simulink model "commhdlQPSKTxRxLoopback"  (R2025b)
settings: Solver=FixedStepDiscrete  StartTime=0.0  StopTime=0.03  RelTol=1e-3
PostLoadFcn:
  | hScopeConfig = get_param([gcs '/Receiver/QPSK Rx/Frequency and Time Synchronizer/Symbol Synchronizer/No HDL/QPSK Receiver Eye Diagram'],'ScopeConfiguration');
  | 
  | hScopeConfig.OpenAtSimulationStart = false;
  | hScopeConfig.Visible = false;
  | SamplesPerSymbol = 4;
  | %UpsamplesRx = 1;
  | clear hScopeConfig
InitFcn:
  | % RxAlign decoder latency (flat_simfix): 41 = netlist value used for HDL; set
  | % rxAlignLat = 25 in the base workspace before a model-level simulation.
  | if ~exist('rxAlignLat','var'), rxAlignLat = uint16(41); end
  | commhdlQPSKTxRxModelInit;
  | % Rate bridge: ADRV9002/Jupiter radio runs at 15.36 MHz = 2x the 7.68 MHz
  | % (4 samples/symbol @ Rsym=1.92 MHz) the QPSK Rx requires. The deployed
  | % Receiver must downsample the ADC stream by 2. UpsamplesRx=1 fed the QPSK
  | % Rx 8 sps (2x-upsampled) and broke symbol sync / the loopback bit check.
  | UpsamplesRx = 1;   %% T8 RATE FIX: rail 15.36e6 == ADC bus rate,
  | %% no ingress decimation (was 2 when the rail sat on the 7.68e6 rung)
  | UpsamplesTx = 1;
  | clear simTimingOffset;
StopFcn:
  | if exist('simTimingOffset','var')
  |   disp('Simulation completed');
  |   %QPSKTxRxVerification;
  | end
undefined symbols (not defined in the file or in its folder): Add, Config, fsym, randsrc, RandStream, Rsym, rxAlignLat, Shift
libraries: hdlsllib x141, simulink x45, dspsigops x30, dsphdlfiltering2 x6, dsphdlsigops2 x4, dsphdlmathfun2 x4, commdigbbndpm3 x4, dspmlti4 x2, commchan3 x1, commrflib2 x1, commcnvcod2 x1
(part 9 of 9)

== matlab function commhdlQPSKTxRxLoopback/TxRxComposite/Transmitter/Input Data/FEC Tx Encoder K5/TxInterleaveK5 ==
  data: codedPair input; dataOut output; infoValid input; beatIdx input; frameValid input; frameStart input
function dataOut = fecTxInterleaveK5(codedPair, infoValid, beatIdx, frameValid, frameStart)
%#codegen
persistent ramA ramB rdBank wptr rrow rcol;
CODED=uint16(49168); COLS=uint16(16); ROWS=uint16(3073);
FILL = logical([1 1 1 1 1 1 1 1 1 0 0 0 0 0 1 1 1 1 0 1 1 1 1 1 0 0 0 1 0 1 1 1 0 0 1 1 0 0 1 0 0 0 0 0 1 0 0 1]);   % 64-bit PN9 filler (T8 fix 6bcaa62)
if isempty(ramA), ramA=fi(zeros(1,49168),0,1,0); ramB=fi(zeros(1,49168),0,1,0); rdBank=false; wptr=uint16(0); rrow=uint16(0); rcol=uint16(0); end
rb=rdBank; w=wptr; rr=rrow; cc=rcol;
dataOut=false;
wr0=uint16(0); wr1=uint16(0); v0=fi(0,0,1,0); v1=fi(0,0,1,0); doW0=false; doW1=false;
if frameValid
  if frameStart, w=uint16(0); rb=~rb; end
  % ---- READ side (previous frame, opposite bank), legacy perm r*COLS+c ----
  % divisionless read address: rr (row 0..ROWS-1) / cc (col 0..COLS-1) are
  % incremental counters, reset on beatIdx==0, advancing +1 row with col carry
  % per in-range beat -- replaces the old per-beat divide-by-ROWS. No divide.
  if beatIdx < CODED
    % precondition: bit-exactness requires a contiguous beatIdx hitting 0 once per
    % frame to re-seed the row/col counters (the old stateless per-beat address
    % arithmetic derived the address from beatIdx alone and needed no such reset).
    if beatIdx == 0, rr = uint16(0); cc = uint16(0); end
    perm = rr*COLS + cc;
    if perm < CODED
      if rb, dataOut = logical(ramB(double(perm)+1)); else, dataOut = logical(ramA(double(perm)+1)); end
    end
    rr = rr + uint16(1);
    if rr == ROWS, rr = uint16(0); cc = cc + uint16(1); end
  else
    dataOut = FILL(double(beatIdx-CODED)+1);   % PN9 filler, beats CODED..2239
  end
  % ---- WRITE side: two coded bits per encoder-advance beat ----
  if infoValid
    if w < CODED, wr0=w; v0=fi(double(codedPair(1)~=0),0,1,0); doW0=true; w=w+uint16(1); end
    if w < CODED, wr1=w; v1=fi(double(codedPair(2)~=0),0,1,0); doW1=true; w=w+uint16(1); end
  end
end
% ---- persist state last (write bank = opposite of read bank) ----
if doW0
  if rb, ramA(double(wr0)+1)=v0; else, ramB(double(wr0)+1)=v0; end
end
if doW1
  if rb, ramA(double(wr1)+1)=v1; else, ramB(double(wr1)+1)=v1; end
end
rdBank=rb; wptr=w; rrow=rr; rcol=cc;

== matlab function commhdlQPSKTxRxLoopback/TxRxComposite/ByteWordBuffer ==
  data: dataIn input; word output; validIn input; popReq input; firstIn input; avail output; readyNext output; wordFirst output
function [word, avail, readyNext, wordFirst] = byteWordBufferBlk(dataIn, validIn, popReq, firstIn)
% Block wrapper around qpskByteWordBufferSkid (unit-tested single source of
% truth); persistent state only. readyNext = the post-update registered
% ready; an external Delay (IC=1) turns it back into the AXIS tready.
% firstIn/wordFirst carry the in-band first-word marker alongside data.
persistent state
if isempty(state)
    state = qpskByteWordBufferSkid();
end
[word, avail, ~, wordFirst, state] = qpskByteWordBufferSkid(state, uint64(dataIn), ...
    logical(validIn), logical(popReq), logical(firstIn));
readyNext = state.readyReg;

== matlab function commhdlQPSKTxRxLoopback/TxRxComposite/ByteSerializer ==
  data: bitIn input; word output; bitValid input; start input; ready input; wordTog output; wordLast output; wordFirst output; bsWv output; bsWl output; bsWcnt output
function [word, wordTog, wordLast, wordFirst, bsWv, bsWl, bsWcnt] = byteSerializerBlk(bitIn, bitValid, start, ready)
% Block wrapper around qpskByteSerializer (unit-tested single source of
% truth); persistent state only. word/wordLast are HELD stable between
% emissions; wordTog flips once per emitted word so the slow->fast rate
% crossing cannot drop or repeat it -- the 30.72M BeatGate edge-detects
% it into exactly one accepted AXIS beat. Dropped words (ready low at
% completion) do not toggle: drop means NO beat, never a stall.
% K5 kit: 382 words/frame = the first 64*382 of
% the 1084 decoded info bits; the trailing 60 are dropped by start-reset.
persistent state tog heldWord heldLast heldFirst firstNext padCount pq0 pq1 pq2 pl0 pl1 pl2 pqn
if isempty(state)
    state = qpskByteSerializer();
    tog = false; heldWord = uint64(0); heldLast = false;
    heldFirst = true; firstNext = true;
    padCount = uint16(0); pqn = uint8(0);
    pq0 = uint64(0); pq1 = uint64(0); pq2 = uint64(0);
    pl0 = false; pl1 = false; pl2 = false;
end
% presentation is decoupled from acceptance (ADI S2MM source style):
% the offered beat must refresh on EVERY completed word or the DMA's
% SYNC_TRANSFER_START gate can wait forever on a frozen user flag /
% accept a stale word. ready at the pin only decides acceptance, so
% the core serializer runs with ready=true and unaccepted beats are
% simply superseded.
bsWcnt = state.wordCnt;   % BS census: words this step's start would abandon
[w, wv, wl, ~, state] = qpskByteSerializer(state, logical(bitIn), ...
    logical(bitValid), logical(start), true, uint16(382));
% PAD (F4) -- frame-length padding for TRUNCATED frames (ledger
% FWD_CRC_REGRESSION_0907 sec 47.5).  A start with 1..WPP-1 words accumulated
% schedules WPP - wordCnt all-zero fillers so the stream stays WPP-word
% aligned; real words completing meanwhile are queued (at most 3) and
% released in order afterwards.
if logical(start) && (padCount == uint16(0)) && ...
   (bsWcnt >= uint16(1)) && (bsWcnt <= uint16(381))
    padCount = uint16(382) - bsWcnt;
end
wR = w; wvR = wv; wlR = logical(wl);
w = uint64(0); wv = false; wl = false;
if padCount ~= uint16(0)
    w = uint64(0); wv = true; wl = (padCount == uint16(1));
    padCount = padCount - uint16(1);
    if wvR
        if pqn == uint8(0)
            pq0 = wR; pl0 = wlR; pqn = uint8(1);
        elseif pqn == uint8(1)
            pq1 = wR; pl1 = wlR; pqn = uint8(2);
        elseif pqn == uint8(2)
            pq2 = wR; pl2 = wlR; pqn = uint8(3);
        end
    end
elseif pqn ~= uint8(0)
    w = pq0; wl = pl0; wv = true;
    pq0 = pq1; pl0 = pl1; pq1 = pq2; pl1 = pl2; pqn = pqn - uint8(1);
    if wvR
        if pqn == uint8(0)
            pq0 = wR; pl0 = wlR; pqn = uint8(1);
        elseif pqn == uint8(1)
            pq1 = wR; pl1 = wlR; pqn = uint8(2);
        elseif pqn == uint8(2)
            pq2 = wR; pl2 = wlR; pqn = uint8(3);
        end
    end
else
    w = wR; wv = wvR; wl = wlR;
end
% BS byte-seam taps on the EMITTED word (rxfix_pad_overlay.m inserts its
% filler/queue arbiter ABOVE this line, so these count fillers too).
bsWv = wv; bsWl = logical(wl);
if wv
    heldWord = w; heldLast = logical(wl); tog = ~tog;
    heldFirst = firstNext; firstNext = logical(wl);
end
word = heldWord; wordTog = tog; wordLast = heldLast; wordFirst = heldFirst;

== matlab function commhdlQPSKTxRxLoopback/Transmitter/QPSK Tx/Bit Packetizer/Data Bits FIFO/MATLAB Function1 ==
  data: wr input; full output; rd input; dataBitsPerPacket parameter
function full = fcn(wr,rd,dataBitsPerPacket)
%#codegen
     
    depth = dataBitsPerPacket*2 - 1;
    persistent count;
    if isempty(count)
        count = fi(0,0,nextpow2(depth),0,hdlfimath);
    end

    if wr
        count(:) = count + 1;
    end
    if rd
        count(:) = count - 1;
    end

    full = (count > depth);

end

== matlab function commhdlQPSKTxRxLoopback/TxRxComposite/ByteRxFifo ==
  data: word input uint64; outWord output uint64; tog input boolean; wLast input boolean; wFirst input boolean; ready input boolean; valid output boolean; outLast output boolean; outFirst output boolean; ovf output uint32
function [outWord, valid, outLast, outFirst, ovf] = byteRxFifo(word, tog, wLast, wFirst, ready)
%#codegen
% 64-deep elastic FIFO: enqueue on serializer toggle edge, dequeue on
% accepted AXIS beat. Drop-newest + count on full (stall > ~19 ms).
% f1536 SOF-prime guard (TXMUX 2026-07-25): valid is presented only after
% ready has been continuously high for 6 cycles, so the axi_dmac S2MM
% per-descriptor SOF prime (5-cycle latency, replicates a HELD beat x5 =
% the W0x5 dup) never sees a held beat during its prime window.
persistent mem memFl wr rd prev ovfCnt rdyRun
if isempty(wr)
    mem = zeros(64,1,'uint64'); memFl = zeros(64,1,'uint8');
    wr = uint16(0); rd = uint16(0); prev = false; ovfCnt = uint32(0);
    rdyRun = uint8(0);
end
if logical(tog) ~= prev
    nxt = uint16(mod(uint32(wr) + 1, 64));
    if nxt == rd
        rd = uint16(mod(uint32(rd) + 1, 64));
        ovfCnt = ovfCnt + uint32(1);
    end
    mem(uint32(wr)+1)   = uint64(word);
    memFl(uint32(wr)+1) = uint8(wLast) + uint8(2)*uint8(wFirst);
    wr = nxt;
end
prev = logical(tog);
valid = (wr ~= rd) && (rdyRun >= uint8(6));
outWord  = mem(uint32(rd)+1);
fl = memFl(uint32(rd)+1);
outLast  = bitand(fl, uint8(1)) ~= uint8(0);
outFirst = bitand(fl, uint8(2)) ~= uint8(0);
if valid && logical(ready)
    rd = uint16(mod(uint32(rd) + 1, 64));
end
if logical(ready)
    if rdyRun < uint8(255), rdyRun = rdyRun + uint8(1); end
else
    rdyRun = uint8(0);
end
ovf = ovfCnt;

== matlab function commhdlQPSKTxRxLoopback/TxRxComposite/Receiver/QPSK Rx/Frequency and Time Synchronizer/Preamble Detector/PdTelemetry ==
  data: validIn input boolean; telI output fixdt(1,16,0); dI input int16; dQ input int16; thrEx input boolean; tRef input uint16; tOff input uint16; done input boolean; newPk input boolean; succ input boolean; sync input boolean; armed input boolean; taRef input uint16; accOff input uint16; fifoEnt input uint16; vPop input boolean; tRefLong input uint32; runMax input uint32; heldTs input uint32; telQ output fixdt(1,16,0)
function [telI, telQ] = pdTelemetry(validIn, dI, dQ, thrEx, tRef, tOff, done, newPk, succ, sync, armed, taRef, accOff, fifoEnt, vPop, tRefLong, runMax, heldTs)
%#codegen
persistent slot symCtr beatCnt aDone aNewPk aThrEx aSync aVPop s0 s1 s2 s3 s4 s5 s6
if isempty(slot)
    slot = uint8(7); symCtr = uint32(0); beatCnt = uint8(0);
    aDone = false; aNewPk = false; aThrEx = false; aSync = false; aVPop = false;
    s0 = uint32(0); s1 = uint32(0); s2 = uint32(0); s3 = uint32(0);
    s4 = uint32(0); s5 = uint32(0); s6 = uint32(0);
end
aDone = aDone || done; aNewPk = aNewPk || newPk; aThrEx = aThrEx || thrEx;
aSync = aSync || sync; aVPop = aVPop || vPop;
if beatCnt < uint8(7), beatCnt = beatCnt + uint8(1); end
if validIn
    symCtr = symCtr + uint32(1);
    flags = uint32(aDone) + bitshift(uint32(aNewPk),1) + bitshift(uint32(succ),2) + ...
            bitshift(uint32(aThrEx),3) + bitshift(uint32(aSync),4) + bitshift(uint32(armed),5);
    s0 = bitor(bitor(bitor(bitshift(uint32(14),28), bitshift(uint32(bitand(tRef,uint16(2047))),17)), ...
         bitshift(uint32(bitand(tOff,uint16(2047))),6)), flags);
    s1 = bitor(bitshift(uint32(reinterpretcast(dI,numerictype(0,16,0))),16), ...
         uint32(reinterpretcast(dQ,numerictype(0,16,0))));
    s2 = bitor(bitor(bitor(bitshift(uint32(bitand(taRef,uint16(2047))),21), ...
         bitshift(uint32(bitand(accOff,uint16(2047))),10)), ...
         bitshift(uint32(bitand(fifoEnt,uint16(511))),1)), uint32(aVPop));
    s3 = tRefLong;
    s4 = runMax;
    s5 = heldTs;
    s6 = bitor(bitor(bitshift(uint32(165),24), bitshift(uint32(bitand(uint16(beatCnt),uint16(7))),21)), ...
         bitand(symCtr,uint32(2097151)));
    aDone = false; aNewPk = false; aThrEx = false; aSync = false; aVPop = false;
    beatCnt = uint8(0);
    slot = uint8(0);
end
switch slot
  case uint8(0), w = s0;
  case uint8(1), w = s1;
  case uint8(2), w = s2;
  case uint8(3), w = s3;
  case uint8(4), w = s4;
  case uint8(5), w = s5;
  case uint8(6), w = s6;
  otherwise,     w = uint32(0);
end
if slot < uint8(7), slot = slot + uint8(1); end
telI = reinterpretcast(uint16(bitshift(w, -16)), numerictype(1,16,0));
telQ = reinterpretcast(uint16(bitand(w, uint32(65535))), numerictype(1,16,0));

== matlab function commhdlQPSKTxRxLoopback/TxRxComposite/Receiver/QPSK Rx/Frequency and Time Synchronizer/Carrier Synchronizer/Loop Filter/LGMux_cs_prop_gain ==
  data: axi input; coeff output; nz output
function [coeff, nz] = cs_prop_gain_mux(axi)
%#codegen
nz = axi ~= uint32(0);
si = bitsliceget(axi, 16, 1);
coeff = reinterpretcast(si, numerictype(0, 16, 16));
end

== matlab function commhdlQPSKTxRxLoopback/TxRxComposite/Receiver/QPSK Rx/Frequency and Time Synchronizer/Carrier Synchronizer/Loop Filter/LGMux_cs_integ_gain ==
  data: axi input; coeff output; nz output
function [coeff, nz] = cs_integ_gain_mux(axi)
%#codegen
nz = axi ~= uint32(0);
si = bitsliceget(axi, 16, 1);
coeff = reinterpretcast(si, numerictype(0, 16, 16));
end

== matlab function commhdlQPSKTxRxLoopback/TxRxComposite/Receiver/QPSK Rx/Frequency and Time Synchronizer/Symbol Synchronizer/Loop Filter/LGMux_ss_prop_gain ==
  data: axi input; coeff output; nz output
function [coeff, nz] = ss_prop_gain_mux(axi)
%#codegen
nz = axi ~= uint32(0);
si = bitsliceget(axi, 24, 1);
coeff = reinterpretcast(si, numerictype(1, 24, 24));
end

== matlab function commhdlQPSKTxRxLoopback/TxRxComposite/Receiver/QPSK Rx/Frequency and Time Synchronizer/Symbol Synchronizer/Loop Filter/LGMux_ss_integ_gain ==
  data: axi input; coeff output; nz output
function [coeff, nz] = ss_integ_gain_mux(axi)
%#codegen
nz = axi ~= uint32(0);
si = bitsliceget(axi, 24, 1);
coeff = reinterpretcast(si, numerictype(1, 24, 24));
end

== matlab function commhdlQPSKTxRxLoopback/TxRxComposite/Receiver/QPSK Rx/Automatic Gain Control/Loop Filter/LGMux_agc_loop_gain ==
  data: axi input; coeff output; nz output
function [coeff, nz] = agc_loop_gain_mux(axi)
%#codegen
nz = axi ~= uint32(0);
si = bitsliceget(axi, 32, 1);
coeff = reinterpretcast(si, numerictype(0, 32, 31));
end

== matlab function commhdlQPSKTxRxLoopback/TxRxComposite/Receiver/QPSK Rx/Frequency and Time Synchronizer/Coarse Frequency Compensator/CFO step change detector/LGMux_cfo_threshold ==
  data: axi input; firePos output; x input; fireNeg output; nz output
function [firePos, fireNeg, nz] = cfo_threshold_mux(axi, x)
%#codegen
nz = axi ~= uint32(0);
si = bitsliceget(axi, 22, 1);
thr = reinterpretcast(si, numerictype(1, 22, 21));
firePos = x > thr;
fireNeg = x < (-thr);
end

== matlab function commhdlQPSKTxRxLoopback/Transmitter/QPSK Tx/Bit Packetizer/Data Bits FIFO/RAM Frame Status Indicator ==
  data: push input; out output; pop input; dataBitsPerPacket parameter
function out = fcn(push,pop,dataBitsPerPacket)

   persistent pushCount popCount frameCount;
   if isempty(pushCount)
       pushCount = fi(0,0,nextpow2(dataBitsPerPacket),0,hdlfimath);
       frameCount = fi(0,0,2,0,hdlfimath);
       popCount = fi(0,0,nextpow2(dataBitsPerPacket),0,hdlfimath);
   end
   
   if (pushCount == dataBitsPerPacket-1) && push
       frameCount(:) = frameCount + 1;
   end
   if (popCount == dataBitsPerPacket-1) && pop
       frameCount(:) = frameCount - 1;
   end

   if push
       if pushCount == dataBitsPerPacket - 1
           pushCount(:) = 0;
       else
           pushCount(:) = pushCount + 1;
       end
   end

   if pop 
       if popCount == dataBitsPerPacket - 1
           popCount(:) = 0;
       else
           popCount(:) = popCount + 1;
       end
   end

   out = frameCount;

end

== matlab function commhdlQPSKTxRxLoopback/TxRxComposite/FrameStatChecksum ==
  data: word input uint64; chk output uint16; wordTog input boolean; strobe input boolean
function chk = frameStatChecksum(word, wordTog, strobe)
%#codegen
% 16-bit running checksum over the delivered RX 64-bit words. On each emitted
% word (wordTog change), the eight bytes of the word are added into a 16-bit
% modular accumulator. chk is COMBINATIONAL (= the accumulated sum of every
% word delivered in the frame completed as of this cycle) so FrameStatProbe,
% latching chk on the SAME strobe edge, captures THIS frame -- no register-to-
% register race / off-by-one (see FRAMESTAT_NOTES.md). Host mirror: for each
% received 64-bit word, add its 8 bytes mod 2^16.
persistent acc prevTog prevStr
if isempty(acc)
    acc = uint16(0); prevTog = false; prevStr = false;
end
chk = acc;
strobeEdge = strobe && ~prevStr;
prevStr = strobe;
if strobeEdge
    acc = uint16(0);
end
if logical(wordTog) ~= prevTog
    s = uint32(0);
    for bpos = 0:8:56
        s = s + uint32(bitand(bitshift(word, -bpos), uint64(255)));
    end
    acc = uint16(mod(uint32(acc) + s, uint32(65536)));
end
prevTog = logical(wordTog);

== matlab function commhdlQPSKTxRxLoopback/TxRxComposite/FrameStatProbe ==
  data: pktCnt input uint32; rec output uint64; rstcsCnt input uint32; runMax input uint32; adcFor input uint32; cfcEst input uint32; chk input uint16; strobe input boolean; stallCnt input uint32; txurCnt input uint32; push output boolean
function [rec, push] = frameStatProbe(pktCnt, rstcsCnt, runMax, adcFor, cfcEst, chk, strobe, stallCnt, txurCnt)
%#codegen
% Latch the 64-bit per-frame status record at the frame strobe. Bit layout:
%   [7:0] frame_seq [8] cs_reset [9] stall_in_frame [10] txur_in_frame
%   [11] sync_low [23:16] corr [31:24] agc [47:32] cfc [63:48] checksum.
% [9]/[10] use the SAME changed-since-last-strobe idiom as cs_reset (the
% free-running counters are the ground truth; comparing latched snapshots
% avoids any cross-rate clear/latch race). See FRAMESTAT_NOTES.md.
persistent rec_r prevRst prevStr prevStall prevTxur
if isempty(rec_r)
    rec_r = uint64(0); prevRst = uint32(0); prevStr = false;
    prevStall = uint32(0); prevTxur = uint32(0);
end
push = false;
% latch once per frame on the strobe rising edge (recStart pulse-or-hold safe)
strobeEdge = strobe && ~prevStr;
prevStr = strobe;
if strobeEdge
    frame_seq = uint64(bitand(pktCnt, uint32(255)));
    cs_reset  = uint64(rstcsCnt ~= prevRst);
    stall_b   = uint64(stallCnt ~= prevStall);
    txur_b    = uint64(txurCnt ~= prevTxur);
    % corr_strength = MSB position (0..32) of the runningMax SI
    corrq = uint32(0);
    for k = 0:31
        if bitshift(runMax, -k) ~= uint32(0)
            corrq = uint32(k + 1);
        end
    end
    sync_low = uint64(corrq < uint32(20));
    corr8 = uint64(bitand(corrq, uint32(255)));
    agc8  = uint64(bitand(bitshift(adcFor, -24), uint32(255)));
    cfc16 = uint64(bitand(bitshift(cfcEst, -5), uint32(65535)));
    chk16 = uint64(chk);
    rec_r = bitor(bitor(bitor(bitor(bitor(bitor(bitor(bitor( ...
        frame_seq, ...
        bitshift(cs_reset, 8)), ...
        bitshift(stall_b, 9)), ...
        bitshift(txur_b, 10)), ...
        bitshift(sync_low, 11)), ...
        bitshift(corr8, 16)), ...
        bitshift(agc8, 24)), ...
        bitshift(cfc16, 32)), ...
        bitshift(chk16, 48));
    prevRst = rstcsCnt;
    prevStall = stallCnt;
    prevTxur  = txurCnt;
    push = true;
end
rec = rec_r;

== matlab function commhdlQPSKTxRxLoopback/TxRxComposite/FrameStatFifo ==
  data: rec input uint64; headLo output uint32; push input boolean; popTok input uint32; headHi output uint32; stat output uint32
function [headLo, headHi, stat] = frameStatFifo(rec, push, popTok)
%#codegen
% 64-deep record FIFO. HEAD = mem(rd). Host: read 0x1D0 (lo), 0x1D4 (hi),
% then write a changed token to 0x1DC to advance. STAT(0x1D8) =
% {ovf[31:16] | level[15:0]}. Drop-newest on full.
persistent mem wr rd ovfCnt prevPop
if isempty(wr)
    mem = zeros(64,1,'uint64'); wr = uint16(0); rd = uint16(0);
    ovfCnt = uint16(0); prevPop = uint32(0);
end
if push
    nxt = uint16(mod(uint32(wr) + 1, 64));
    if nxt == rd
        if ovfCnt < uint16(65535), ovfCnt = ovfCnt + uint16(1); end
    else
        mem(uint32(wr)+1) = rec;
        wr = nxt;
    end
end
if popTok ~= prevPop
    if wr ~= rd, rd = uint16(mod(uint32(rd) + 1, 64)); end
end
prevPop = popTok;
head = mem(uint32(rd)+1);
headLo = uint32(bitand(head, uint64(4294967295)));
headHi = uint32(bitshift(head, -32));
level  = uint32(mod(uint32(wr) - uint32(rd) + 64, 64));
stat   = bitor(bitshift(uint32(ovfCnt), 16), level);

== matlab function commhdlQPSKTxRxLoopback/TxRxComposite/FrameStatWordCnt ==
  data: vld input boolean; cnt output uint32; rdy input boolean
function cnt = frameStatWordCnt(vld, rdy)
%#codegen
% free-running 32-bit accepted-word counter (byte_rx_valid && byte_rx_ready).
% Wraps mod 2^32 (uint32 native wrap is not guaranteed saturation-free in
% MLFB codegen defaults, so wrap explicitly).
persistent c
if isempty(c)
    c = uint32(0);
end
cnt = c;
if vld && rdy
    if c == uint32(4294967295)
        c = uint32(0);
    else
        c = c + uint32(1);
    end
end

== matlab function commhdlQPSKTxRxLoopback/TxRxComposite/FrameStatStallCnt ==
  data: vld input boolean; cnt output uint32; rdy input boolean
function cnt = frameStatStallCnt(vld, rdy)
%#codegen
% free-running 32-bit STALL-cycle counter (byte_rx_valid && ~byte_rx_ready):
% each count is one cycle the DMAC backpressured an offered byte_rx beat.
% Wraps mod 2^32 explicitly (same idiom as FrameStatWordCnt).
persistent c
if isempty(c)
    c = uint32(0);
end
cnt = c;
if vld && ~rdy
    if c == uint32(4294967295)
        c = uint32(0);
    else
        c = c + uint32(1);
    end
end

== matlab function commhdlQPSKTxRxLoopback/TxRxComposite/FrameStatTxUrCnt ==
  data: ur input boolean; cnt output uint32
function cnt = frameStatTxUrCnt(ur)
%#codegen
% free-running 32-bit TX-underrun EVENT counter: one count per
% ByteBitShifter underflow reload (modulator starved -> zeros aired for
% the frame remainder). Wraps mod 2^32 explicitly (FrameStatWordCnt idiom).
persistent c
if isempty(c)
    c = uint32(0);
end
cnt = c;
if ur
    if c == uint32(4294967295)
        c = uint32(0);
    else
        c = c + uint32(1);
    end
end

== matlab function commhdlQPSKTxRxLoopback/TxRxComposite/Receiver/QPSK Rx/BeatObs ==
  data: dOut input; dbgI1 output; sOut input; vOut input; decis input; rhc input; pushc input; popc input; dbgQ1 output
function [dbgI1, dbgQ1] = fcn(dOut, sOut, vOut, decis, rhc, pushc, popc)
%#codegen
fill8 = bitand(uint32(pushc) - uint32(popc), uint32(255));
acc = uint32(dOut ~= 0);
acc = acc + uint32(2)  * uint32(sOut ~= 0);
acc = acc + uint32(4)  * uint32(vOut ~= 0);
acc = acc + uint32(8)  * uint32(decis(1) ~= 0);
acc = acc + uint32(16) * uint32(decis(2) ~= 0);
acc = acc + uint32(32) * bitand(uint32(rhc), uint32(3));
acc = acc + uint32(256) * fill8;
qcc = bitand(uint32(pushc), uint32(255)) + uint32(256) * bitand(uint32(popc), uint32(255));
dbgI1 = uint16(bitand(acc, uint32(65535)));
dbgQ1 = uint16(bitand(qcc, uint32(65535)));

== matlab function commhdlQPSKTxRxLoopback/TxRxComposite/Receiver/QPSK Rx/FixCtlDec ==
  data: ctl input; enContract output; enSerAnchor output; enGridPace output; w1Freeze output; sroSign output
function [enContract, enSerAnchor, enGridPace, w1Freeze, sroSign] = fcn(ctl)
%#codegen
enContract  = bitand(uint32(ctl), uint32(1)) ~= uint32(0);
enSerAnchor = bitand(uint32(ctl), uint32(2)) ~= uint32(0);
enGridPace  = bitand(uint32(ctl), uint32(4)) ~= uint32(0);
w1Freeze    = bitand(uint32(ctl), uint32(16)) ~= uint32(0);
sroSign     = bitand(uint32(ctl), uint32(32)) ~= uint32(0);

== matlab function commhdlQPSKTxRxLoopback/TxRxComposite/Receiver/QPSK Rx/BfTagGen ==
  data: vin input; tag output; sin input
function tag = fcn(vin, sin)
%#codegen
persistent t
if isempty(t), t = uint16(0); end
if vin
  if sin
    t = uint16(0);
  elseif t >= uint16(24607)
    t = uint16(0);
  else
    t = t + uint16(1);
  end
end
tag = t;

== matlab function commhdlQPSKTxRxLoopback/Receiver/QPSK Rx/Frequency and Time Synchronizer/Packet Controller/sample discard controller ==
  data: dataIn input; validIn input; dataOut output; startIn input; endIn input; startOut output; endOut output; validOut output
function [dataOut,startOut,endOut,validOut] = controller(dataIn,validIn,startIn,endIn)
%#codegen

   persistent active dataOutReg validOutReg startOutReg endOutReg;
   if isempty(active)
      active  = false;
      dataOutReg = cast(0,'like',dataIn);
      validOutReg = false;
      startOutReg = false;
      endOutReg = false;
   end
   
   dataOut = dataOutReg;
   validOut = validOutReg;
   startOut = startOutReg;
   endOut = endOutReg;
   
   startOutReg = startIn;
   endOutReg = endIn;
   
   if startIn
       active = true;
   end
   
   if active
       dataOutReg(:) = dataIn;
       validOutReg = validIn;
   else
       dataOutReg(:) = 0;
       validOutReg = false;
   end
   
   if endIn
       if active 
           endOutReg = true;
       else
           endOutReg = false;
       end
       active = false;
   end
end

== matlab function commhdlQPSKTxRxLoopback/TxRxComposite/Receiver/QPSK Rx/BfContract ==
  data: tagd input; startSel output; vout input; legacyStart input; enContract input; violCount output; violLatch output
function [startSel, violCount, violLatch] = fcn(tagd, vout, legacyStart, enContract)
%#codegen
persistent prev cnt lat started K kvalid enPrev voutPrev
if isempty(prev), prev = uint16(0); cnt = uint32(0); lat = uint32(0); started = false; K = uint16(0); kvalid = false; enPrev = false; voutPrev = false; end
% v3 EDGE QUALIFIER (pcFirstBit): vout is a 2-beat LEVEL per coded bit; act only
% on the first beat (tag-advance beat) -- fixes the 2-beat start pulse (the v1/v2
% +1-bit framing shift = A90B79F1) AND the per-bit false violation counting.
vEdge = vout && ~voutPrev;
voutPrev = logical(vout);
% v2 SELF-CALIBRATING ANCHOR: on enContract rising edge, forget K; latch K = tag
% at the next LEGACY frame start (alignment known-good right after bring-up).
if enContract && ~enPrev, kvalid = false; end
enPrev = enContract;
if enContract && ~kvalid && (legacyStart ~= 0) && vEdge
  K = tagd; kvalid = true;
end
% continuity check (ALWAYS ON, read-only)
if vEdge
  if started
    expd = prev + uint16(1);
    if expd >= uint16(24608), expd = uint16(0); end
    if tagd ~= expd
      cnt = cnt + uint32(1);
      d = int32(tagd) - int32(expd);
      lat = bitor(bitshift(bitand(uint32(d), uint32(65535)), 16), uint32(prev));
    end
  end
  started = true;
  prev = tagd;
end
% contract frame start: tag==K (calibrated) on a valid beat; legacy until calibrated
cs = vEdge && kvalid && (tagd == K);
if enContract && kvalid
  startSel = cs;
else
  startSel = legacyStart ~= 0;
end
violCount = cnt;
violLatch = lat;

== matlab function commhdlQPSKTxRxLoopback/TxRxComposite/Receiver/QPSK Rx/QPSK Demodulator/Serializer/BfSerMux ==
  data: c input; y output; anchor input
function y = fcn(c, anchor)
%#codegen
if anchor
  y = uint8(0);
else
  y = uint8(c);
end

== matlab function commhdlQPSKTxRxLoopback/TxRxComposite/Receiver/QPSK Rx/Frequency and Time Synchronizer/Symbol Synchronizer/Rate Handle/BfGridPace ==
  data: c input; y output; en input
function y = fcn(c, en)
%#codegen
persistent a
if isempty(a), a = uint8(0); end
% absolute pacer: counts EVERY beat unconditionally
if a >= uint8(3), a = uint8(0); else, a = a + uint8(1); end
if en
  y = a;
else
  y = uint8(c);
end

== matlab function commhdlQPSKTxRxLoopback/TxRxComposite/Receiver/QPSK Rx/Frequency and Time Synchronizer/RxW1Census ==
  data: occ input; witA output; pushPtr input; popPtr input; popEmpty input; pushFull input; vSS input; vRH input; vCFC input; vCS input; vPD input; vPC input; freeze input; witB output; cSS output; cRH output; cCFC output; cCS output; cPD output; cPC output
function [witA, witB, cSS, cRH, cCFC, cCS, cPD, cPC] = fcn(occ, pushPtr, popPtr, popEmpty, pushFull, vSS, vRH, vCFC, vCS, vPD, vPC, freeze)
%#codegen
persistent poe pof lSS lRH lCFC lCS lPD lPC sA sB sSS sRH sCFC sCS sPD sPC
if isempty(poe)
  poe = uint16(0); pof = uint16(0);
  lSS = uint32(0); lRH = uint32(0); lCFC = uint32(0); lCS = uint32(0); lPD = uint32(0); lPC = uint32(0);
  sA = uint32(0); sB = uint32(0);
  sSS = uint32(0); sRH = uint32(0); sCFC = uint32(0); sCS = uint32(0); sPD = uint32(0); sPC = uint32(0);
end
% outputs = the shadow registered on the PREVIOUS enb beat (assign witA = sA)
witA = sA; witB = sB;
cSS = sSS; cRH = sRH; cCFC = sCFC; cCS = sCS; cPD = sPD; cPC = sPC;
% wA/wB: wires off THIS beat inputs and the PRE-edge edge counters
wA = bitor(bitor(bitshift(bitand(uint32(occ), uint32(63)), 10), bitshift(bitand(uint32(pushPtr), uint32(31)), 5)), bitand(uint32(popPtr), uint32(31)));
wB = bitor(bitshift(uint32(pof), 16), uint32(poe));
% freeze is a LEVEL: hold every shadow while the live counters keep running
if ~freeze
  sA = wA; sB = wB;
  sSS = lSS; sRH = lRH; sCFC = lCFC; sCS = lCS; sPD = lPD; sPC = lPC;
end
% live counters, incremented AFTER the capture; all of them WRAP
if popEmpty
  if poe == uint16(65535), poe = uint16(0); else, poe = poe + uint16(1); end
end
if pushFull
  if pof == uint16(65535), pof = uint16(0); else, pof = pof + uint16(1); end
end
if vSS
  if lSS == uint32(4294967295), lSS = uint32(0); else, lSS = lSS + uint32(1); end
end
if vRH
  if lRH == uint32(4294967295), lRH = uint32(0); else, lRH = lRH + uint32(1); end
end
if vCFC
  if lCFC == uint32(4294967295), lCFC = uint32(0); else, lCFC = lCFC + uint32(1); end
end
if vCS
  if lCS == uint32(4294967295), lCS = uint32(0); else, lCS = lCS + uint32(1); end
end
if vPD
  if lPD == uint32(4294967295), lPD = uint32(0); else, lPD = lPD + uint32(1); end
end
if vPC
  if lPC == uint32(4294967295), lPC = uint32(0); else, lPC = lPC + uint32(1); end
end

== matlab function commhdlQPSKTxRxLoopback/TxRxComposite/Receiver/QPSK Rx/Frequency and Time Synchronizer/Symbol Synchronizer/Rate Handle/RxSteer ==
  data: validIn input; skipEn output; popNom input; occ input; phase2 input; pcEnd input; sroSign input; extraEn output; r4Wit output; r4Extras output; sroMode output
function [skipEn, extraEn, r4Wit, r4Extras, sroMode] = fcn(validIn, popNom, occ, phase2, pcEnd, sroSign)
%#codegen
persistent win wslot skipDone extraDone skipArm extraArm frames skips opens extras pcPend
if isempty(win)
  win = false; wslot = uint8(0); skipDone = false; extraDone = false; pcPend = uint16(0);
  skipArm = false; extraArm = false; frames = uint8(0);
  skips = uint16(0); opens = uint16(0); extras = uint16(0);
end
% wires off the PRE-edge registers (the injector's assign lines)
locked  = frames == uint8(8);
occLe8  = occ <= uint8(8);
occGe24 = occ >= uint8(24);
skipEn  = skipArm;
extraEn = extraArm;
doSkip  = skipArm & popNom;
doExtra = extraArm & validIn & phase2 & sroSign;
r4Wit    = bitor(bitor(bitshift(uint32(locked), 31), bitshift(uint32(skips), 15)), uint32(opens));
r4Extras = uint32(extras);
sroMode  = bitor(bitshift(uint32(extraArm), 1), uint32(sroSign));
% (f) THE REGISTERED DECISION -- pre-edge state only, applied at the end
if doSkip
  nSkipArm = false;
else
  nSkipArm = locked & win & occLe8 & ~skipDone & (wslot <= uint8(12));
end
if doExtra
  nExtraArm = false;
else
  nExtraArm = locked & win & occGe24 & ~extraDone & (wslot <= uint8(12)) & sroSign;
end
% (b) LOCK: eight pcEnd pulses since reset
if pcEnd && ~locked
  frames = frames + uint8(1);
end
% (c) the skip / the extra, and their witnesses (skips/extras/opens WRAP;
%     frames does NOT -- it is capped by its own lock gate at 8, never 15)
if doSkip
  if skips == uint16(65535), skips = uint16(0); else, skips = skips + uint16(1); end
  skipDone = true;
end
if doExtra
  if extras == uint16(65535), extras = uint16(0); else, extras = extras + uint16(1); end
  extraDone = true;
end
% (d) one window slot per NOMINAL pop opportunity, taken or not
if win && popNom
  if wslot >= uint8(13)
    win = false;
  else
    wslot = wslot + uint8(1);
  end
end
% (e) a pcEnd OPENS the window -- last, so it wins over (c) and (d).
% 24534 > 0 (sps 2): open it 24534 nominal pops after pcEnd instead,
% i.e. SlotsPerFrame - lead before the NEXT pcEnd, so the skip/extra lands in the
% filler+preamble of the frame entering the ring and not in its data (see overlay header).
openNow = false;
if pcEnd
  if uint16(24534) == uint16(0), openNow = true; else, pcPend = uint16(24534); end
elseif pcPend > uint16(0) && popNom
  pcPend = pcPend - uint16(1);
  if pcPend == uint16(0), openNow = true; end
end
if openNow
  win = true; wslot = uint8(0); skipDone = false; extraDone = false;
  if opens == uint16(32767), opens = uint16(0); else, opens = opens + uint16(1); end
end
skipArm = nSkipArm;
extraArm = nExtraArm;

== matlab function commhdlQPSKTxRxLoopback/TxRxComposite/Receiver/QPSK Rx/Frequency and Time Synchronizer/Preamble Detector/PdPopIndex ==
  data: delay8Out input; pop output; numEntries input
function pop = fcn(delay8Out, numEntries)
%#codegen
% RXFIX_R1: the realignment FIFO is popped by OCCUPANCY, not by enb ticks.
% numEntries is the registered occupancy and the ring guard bounds it to
% 0..24634, so ==24634 is exactly "full"; popping on push & full fixes the
% data delay at 24634 VALIDS (one frame of slots) for ever.  Stateless on purpose (see the
% overlay header): no persistents => no HDL Coder input delay-match register
% on this DATA-PATH signal.
pop = delay8Out & (numEntries == uint16(24634));

== matlab function commhdlQPSKTxRxLoopback/TxRxComposite/BsSerCensus ==
  data: wv input; sWords output; wl input; wcnt input; sstart input; sStarts output; sLasts output; sTrunc output; sOrd output
function [sWords, sStarts, sLasts, sTrunc, sOrd] = fcn(wv, wl, wcnt, sstart)
%#codegen
% RXFIX_BS, serializer half.  Every counter WRAPS (read as deltas); the three
% order statistics and q24 SATURATE.  tMin resets to WPP and tMax to 0 so the
% first event sets both.  MATLAB integer arithmetic SATURATES where the RTL
% wraps, so each wrapping increment is written out explicitly.
persistent cWords cStarts cLasts cTrunc tLast tMin tMax q24
if isempty(cWords)
  cWords = uint32(0); cStarts = uint32(0); cLasts = uint16(0); cTrunc = uint16(0);
  tLast = uint16(0); tMin = uint16(382); tMax = uint16(0); q24 = uint16(0);
end
if wv
  if cWords == uint32(4294967295), cWords = uint32(0); else, cWords = cWords + uint32(1); end
  if wl
    if cLasts == uint16(65535), cLasts = uint16(0); else, cLasts = cLasts + uint16(1); end
  end
end
if sstart
  if cStarts == uint32(4294967295), cStarts = uint32(0); else, cStarts = cStarts + uint32(1); end
  % a start with 1..WPP-1 words accumulated is a TRUNCATED frame: those words never
  % reach a wordLast.  wcnt == 0 is a clean boundary and wcnt == WPP cannot occur
  % (the counter is cleared when it reaches WPP).
  if (wcnt >= uint16(1)) && (wcnt <= uint16(381))
    wc8 = wcnt;
    if cTrunc == uint16(65535), cTrunc = uint16(0); else, cTrunc = cTrunc + uint16(1); end
    tLast = wc8;
    if wc8 < tMin, tMin = wc8; end
    if wc8 > tMax, tMax = wc8; end
    dfc = uint16(382) - wc8;
    if (dfc == uint16(24)) || (dfc == uint16(48)) || (dfc == uint16(72)) || (dfc == uint16(96)) || (dfc == uint16(120)) || (dfc == uint16(144)) || (dfc == uint16(168)) || (dfc == uint16(192)) || (dfc == uint16(216)) || (dfc == uint16(240)) || (dfc == uint16(264)) || (dfc == uint16(288)) || (dfc == uint16(312)) || (dfc == uint16(336)) || (dfc == uint16(360))
      if q24 ~= uint16(31), q24 = q24 + uint16(1); end
    end
  end
end
sWords = cWords; sStarts = cStarts; sLasts = cLasts; sTrunc = cTrunc;
% sOrd = {tLast, tMin, tMax, q24} (9/9/9/5 bits) -- one 32-bit crossing instead of four.
sOrd = bitor(bitor(bitshift(uint32(tLast), 23), bitshift(uint32(tMin), 14)), ...
            bitor(bitshift(uint32(tMax), 5), uint32(q24)));

== matlab function commhdlQPSKTxRxLoopback/TxRxComposite/BsSeamCensus ==
  data: sWords input; cWords output; sStarts input; sLasts input; sTrunc input; sOrd input; tog input; wFirst input; valid input; ready input; fixctl input; cStarts output; cPush output; cPop output; cDrop output; cMarks output; cEvt output; cCnt output
function [cWords, cStarts, cPush, cPop, cDrop, cMarks, cEvt, cCnt] = fcn(sWords, sStarts, sLasts, sTrunc, sOrd, tog, wFirst, valid, ready, fixctl)
%#codegen
% RXFIX_BS, FIFO half + packing + shadow.  STATEMENT ORDER IS THE RTL'S, not
% the natural one (rh_w1_census / RxW1Census precedent): `assign bus = {s7..s0}`
% means the value visible during beat k is the shadow CAPTURED at edge k-1, and
% the shadow takes the PRE-increment counters.  So: outputs first, then the
% capture, then the increments.  freeze is a LEVEL -- the shadows hold while the
% live counters keep running.
persistent prevTog occ lPush lPop lDrop lMarkP dropRun dropMax s0 s1 s2 s3 s4 s5 s6 s7
if isempty(prevTog)
  prevTog = false; occ = uint16(0);
  lPush = uint32(0); lPop = uint32(0); lDrop = uint32(0); lMarkP = uint16(0);
  dropRun = uint16(0); dropMax = uint16(0);
  s0 = uint32(0); s1 = uint32(0); s2 = uint32(0); s3 = uint32(0);
  s4 = uint32(0); s5 = uint32(0); s6 = uint32(0); s7 = uint32(0);
end
cWords = s0; cStarts = s1; cPush = s2; cPop = s3;
cDrop = s4; cMarks = s5; cEvt = s6; cCnt = s7;
% the three seam events, from the BRAM drop-in's PORTS and its own rules
% (docs/evidence/sp3/BYTERXFIFO_DROPIN.md): push = tog edge, pop = valid_i &&
% ready_1, drop = the drop-OLDEST test wr+1 == rd_after_pop on the occupancy.
push = (logical(tog) ~= prevTog);
pop  = logical(valid) && logical(ready);   % HDL Coder pads `ready` by 4 = the drop-in's ready_1
pN = uint16(0); if pop, pN = uint16(1); end
% + DEPTH before the subtract: MATLAB unsigned arithmetic SATURATES at 0 where
% the RTL pointer wraps, and this test is exactly about the wrap.
drop = push && (bitand(occ + uint16(8192) - pN, uint16(8191)) == uint16(8191));
dN = uint16(0); if drop, dN = uint16(1); end
uN = uint16(0); if push, uN = uint16(1); end
% the eight words as wires off THIS beat's inputs and the PRE-edge counters
w0 = sWords;
w1 = sStarts;
w2 = lPush;
w3 = lPop;
w4 = lDrop;
w5 = bitor(bitshift(uint32(sLasts), 16), uint32(lMarkP));
% w6 = {tLast, tMin, tMax, dropMax}: sOrd carries the first three, q24 is in its
% low 5 bits and belongs to w7.
w6 = bitor(bitand(sOrd, uint32(4294967264)), uint32(dropMax));
w7 = bitor(bitshift(uint32(sTrunc), 16), bitshift(bitand(sOrd, uint32(31)), 8));
% freeze = fixctl bit 4 (header note 4), the same level W1 shadows behind
if bitand(uint32(fixctl), uint32(16)) == uint32(0)
  s0 = w0; s1 = w1; s2 = w2; s3 = w3; s4 = w4; s5 = w5; s6 = w6; s7 = w7;
end
% live counters, incremented AFTER the capture; the 32/16-bit ones WRAP
if push
  if lPush == uint32(4294967295), lPush = uint32(0); else, lPush = lPush + uint32(1); end
  if wFirst
    if lMarkP == uint16(65535), lMarkP = uint16(0); else, lMarkP = lMarkP + uint16(1); end
  end
  % drop implies push in this RTL, so the run length advances on pushes only
  if drop
    if dropRun ~= uint16(31), dropRun = dropRun + uint16(1); end
  else
    dropRun = uint16(0);
  end
  if dropRun > dropMax, dropMax = dropRun; end
end
if pop
  if lPop == uint32(4294967295), lPop = uint32(0); else, lPop = lPop + uint32(1); end
end
if drop
  if lDrop == uint32(4294967295), lDrop = uint32(0); else, lDrop = lDrop + uint32(1); end
end
occ = bitand(occ + uint16(8192) + uN - pN - dN, uint16(8191));
prevTog = logical(tog);

== matlab function commhdlQPSKTxRxLoopback/VGen ==
  data: tick input; v output
function v = vgen(tick)
persistent p
if isempty(p), p=false; end
p = ~p;
v = p && logical(tick);

== matlab function commhdlQPSKTxRxLoopback/ByteSrc ==
  data: ready input; data output; nWords input; valid output; first output
function [data, valid, first] = src(ready, nWords)
persistent idx
if isempty(idx), idx = uint32(1); end
data = uint64(idx);
valid = true;
first = (idx == uint32(1));
if ready
    idx = idx + 1;
    if idx > uint32(nWords), idx = uint32(1); end
end

== matlab function commhdlQPSKTxRxLoopback/Receiver/QPSK Rx/Frequency and Time Synchronizer/Symbol Synchronizer/Interpolation Control ==
  data: mu output; Delta input; Underflow output
function [mu,Underflow] = Interpolation_ctrl(Delta)
% Implementation of modulo-1 counter for interpolation control listed in
% Figure 8.4.19 of "Digital Communications - A Discrete-Time Approach"
% by Michael Rice. See design details in Chapter 8.4.3 of the same book.
% 
% Input:
%   Delta - Loop filter output. If loop is in lock, delta would be small
% Output:
%   Underflow - Indicator of counter underflow. This is the strobe signal
%               for downstream processing
%   mu - Difference between actual sampling instant and the optimal instant,
%        between zero and one
%#codegen

% countReg - Counter value delayed by 1 sample
% muReg - The estimated timing error normalized by half QPSK symbols

   mask = fi(1-2^(-10),1,11,10);
   
   persistent countReg underflowReg muReg;
   if isempty(countReg)
       countReg  = fi(0,1,11,10);
       muReg = fi(0,1,11,10);
       underflowReg = false;
   end
   
   
   Underflow = underflowReg;
   mu = muReg;   
   
   
      % T8.4 anti-wedge clamp: if Delta <= -0.125 the decrementing counter
   % never underflows (strobes stop FOREVER -- Class-4 wedge / Class-1
   % episode mechanism; see tb_timing_wedge.v). Bound Delta so the
   % counter always decrements by >= 1 LSB.
   wlim = fi(511/1024,1,11,10);
   if Delta > wlim
       Delta = wlim;
   elseif Delta < -wlim
       Delta = fi(-511/1024,1,11,10);
   end
   counter = bitand(mask,countReg)-Delta-fi(0.5,1,11,10); % decrementing counter
   
   % if countReg is a nonnegative number,
   % then mod(countReg,1) equals the fractional part of countReg
   if counter < 0
       underflowReg = true;
       muReg = bitshift(bitand(mask,countReg),1);
       countReg = fi(counter+1,1,11,10);% create underflow to counter
   else
       underflowReg = false;
       countReg = fi(counter,1,11,10);
   end
   


end

== matlab function commhdlQPSKTxRxLoopback/Receiver/QPSK Rx/Frequency and Time Synchronizer/Preamble Detector/Correlator/ThresholdLimiter ==
  settings: fimath=hdlfimath
  data: x input; y output
function y = applyLowerLimit(x)
    % Apply a lower limit to the threshold.
    %#codegen
    
    % Threshold is computed by summing across 63 samples.
    % Set lower limit to be equivalent of all 63 samples
    % having their LSB set to 1 and all others set to 0. 
    lowerLimit = cast(0.01, 'like', x);
    
    if x < lowerLimit
        y = lowerLimit;
    else
        y = x;
    end
end

== matlab function commhdlQPSKTxRxLoopback/Transmitter/Input Data/Message Generator/MATLAB Function ==
  data: enable input; reset input; out output; start output; stop output; valid output; count_out output; msg_count_out output
function [out, start, stop, valid, count_out, msg_count_out] = msggen(enable, reset)

persistent indexCount;
persistent toggle;
persistent msgCount;
persistent msgCountAll;
persistent msgCountBitIndex;

if isempty(indexCount) || isempty(toggle) || isempty(msgCount) || isempty(msgCountBitIndex) || isempty(msgCountAll)
    indexCount = uint32(0);
    msgCount = uint32(1);
    msgCountAll = uint32(1);
    msgCountBitIndex = uint8(0);
    toggle = false;
end

%% Constants
strAscii = dec2bin('ADI Hello World', 8);
msgarray = reshape(strAscii', [1, numel(strAscii)]);
msgbits = logical(msgarray - 48);
msgbitsLen = length(msgbits);

fullMessageLen = uint32(2240-1); % Need the -1 to eat the feedback delay

% Bit counter
% N = 8;% 8-bit counter
% mask = uint32(2^N - 1);
% for k = 1:300
%     msgCount = bitand(msgCount + uint32(1), mask);   % wraps 255 -> 0
% end

%% Logic
if enable && ~reset
    % Set out data
    if indexCount < msgbitsLen % Insert msg
        out = msgbits(indexCount + 1);
        msgCountBitIndex = uint8(0);
    else % Zero padding: varying filler (counter digit + toggle bits)
        % caused periodic false-lock error bursts in the deployed BIST;
        % zero-padded payload matches the verified host golden structure.
        out = false;
        msgCountBitIndex = uint8(0);
    end

    % Flags
    start = indexCount == uint32(0);
    stop = indexCount == fullMessageLen;
    valid = true;

    % Counters
    if fullMessageLen == indexCount
        if msgCount >= 9
            msgCount = uint32(1);
        else
            msgCount = msgCount +  1;
            msgCountAll = msgCountAll + 1;
        end
    end
    if indexCount <= fullMessageLen
        indexCount = indexCount + 1;
    end

else % Enable == false

    if reset
        indexCount = uint32(0);
        % msgCount = uint32(0);
        msgCountBitIndex = uint8(0);
        toggle = false;
    end
    out = false;
    start = false;
    stop = false;
    valid = false;
end

if isempty(indexCount)
    count_out = uint32(0);
else
    count_out = indexCount;
end

msg_count_out = msgCountAll;
